simulink model "QuadcopterPID_Prop_Force_Thrust"  (R2026b)
settings: Solver=VariableStepAuto  StopTime=30  MaxStep=1e-2
undefined symbols (not defined in the file or in its folder): g, kT, M
libraries: slpidlib x1
settings Model: Creator=Aorus PC  LastModifiedBy=Ninad
settings OptimizationCC: ReuseModelBlockBuffer=off
settings SimscapeCC: SimscapeUseEnergyAccounting=off

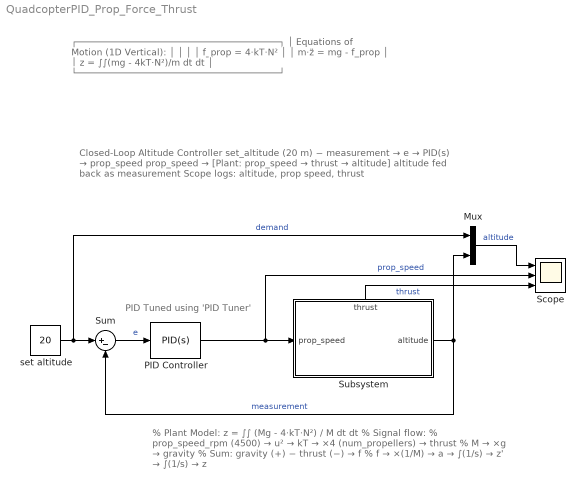
== system QuadcopterPID_Prop_Force_Thrust ==
  note: PID Tuned using 'PID Tuner'
  note: ┌──────────────────────────────────────┐
      | │  Equations of Motion (1D Vertical):  │
      | │                                      │
      | │  f_prop = 4·kT·N²                    │
      | │  m·z̈ = mg - f_prop                  │
      | │  z = ∫∫(mg - 4kT·N²)/m dt dt        │
      | └──────────────────────────────────────┘
  note: Closed-Loop Altitude Controller
      | set_altitude (20 m) − measurement → e → PID(s) → prop_speed
      | prop_speed → [Plant: prop_speed → thrust → altitude]
      | altitude fed back as measurement
      | Scope logs: altitude, prop speed, thrust
  note: % Plant Model: z = ∫∫ (Mg - 4·kT·N²) / M  dt dt
      | % Signal flow:
      | %   prop_speed_rpm (4500) → u² → kT → ×4 (num_propellers) → thrust
      | %   M → ×g → gravity
      | %   Sum: gravity (+) − thrust (−) → f
      | %   f → ×(1/M) → a → ∫(1/s) → z' → ∫(1/s) → z
  Mux : Mux  Inputs=2
  PID Controller : slpidlib/PID Controller  Controller=PID  Form=Parallel  TimeDomain=Continuous-time  UseExternalTs=off  SampleTime=-1  IntegratorMethod=Forward Euler  FilterMethod=Forward Euler  ControllerParametersSource=internal  P=200  I=50  UseKiTs=off  D=150  UseExternalDerivativeSource=off  N=10  UseFilter=on  TunerSelectOption=Transfer Function Based (PID Tuner App)  InitialConditionSource=internal  InitialConditionForIntegrator=4500  InitialConditionForFilter=0  DifferentiatorICPrevScaledInput=0  ExternalReset=none  TrackingMode=off  Kt=1  LimitOutput=on  SatLimitsSource=internal  UpperSaturationLimit=1e4  LowerSaturationLimit=0  LinearizeAsGain=on  AntiWindupMode=back-calculation  Kb=1  LimitIntegrator=on  UpperIntegratorSaturationLimit=1e4  LowerIntegratorSaturationLimit=0  POutMin=[]  POutMax=[]  IOutMin=[]  IOutMax=[]  DOutMin=[]  DOutMax=[]  NOutMin=[]  NOutMax=[]  SumOutMin=[]  SumOutMax=[]  SaturationOutMin=[]  SaturationOutMax=[]  PParamMin=[]  PParamMax=[]  IParamMin=[]  IParamMax=[]  DParamMin=[]  DParamMax=[]  NParamMin=[]  NParamMax=[]  KbParamMin=[]  KbParamMax=[]  KtParamMin=[]  KtParamMax=[]  KbOutMin=[]  KbOutMax=[]  KtOutMin=[]  KtOutMax=[]  IntegratorOutMin=[]  IntegratorOutMax=[]  FilterOutMin=[]  FilterOutMax=[]  SumI1OutMin=[]  SumI1OutMax=[]  SumI2OutMin=[]  SumI2OutMax=[]  SumI3OutMin=[]  SumI3OutMax=[]  SumI4OutMin=[]  SumI4OutMax=[]  SumDOutMin=[]  SumDOutMax=[]  DifferentiatorOutMin=[]  DifferentiatorOutMax=[]  FilterDiffOutCoefMin=[]  FilterDiffOutCoefMax=[]  ReciprocalOutMin=[]  ReciprocalOutMax=[]  SumDenOutMin=[]  SumDenOutMax=[]  SumNumOutMin=[]  SumNumOutMax=[]  DivideOutMin=[]  DivideOutMax=[]  UdiffTsProdOutMin=[]  UdiffTsProdOutMax=[]  NTsProdOutMin=[]  NTsProdOutMax=[]  UintegralTsProdOutMin=[]  UintegralTsProdOutMax=[]  UngainTsProdOutMin=[]  UngainTsProdOutMax=[]  ClampingZeroOutDataTypeStr=Inherit: Inherit via back propagation  ClampingZeroOutMin=[]  ClampingZeroOutMax=[]  FilterDenConstantOutDataTypeStr=Inherit: Inherit via back propagation  FilterDenConstantOutMin=[]  FilterDenConstantOutMax=[]  PCopyOutDataTypeStr=Inherit: Inherit via back propagation  PCopyOutMin=[]  PCopyOutMax=[]  NCopyOutDataTypeStr=Inherit: Inherit via back propagation  NCopyOutMin=[]  NCopyOutMax=[]  IntegratorContinuousStateAttributes=''  IntegratorStateMustResolveToSignalObject=off  IntegratorRTWStateStorageClass=Auto  FilterContinuousStateAttributes=''  FilterStateMustResolveToSignalObject=off  FilterRTWStateStorageClass=Auto  ParallelPVariant=InternalParameters  IdealPVariant=Disabled  IVariant=InternalParameters  DVariant=InternalParameters  IntegratorVariant=Continuous  SatVariant=Enabled  AWVariant=BackCalculation  PCopyVariant=Disabled  TRVariant=Disabled  FdbkBlocksVariant=Forward  IdealPFdbkVariant=Disabled  SatFdbkVariant=Disabled  DerivativeFilterVariant=ContFilter  NVariant=InternalParameters  NCopyVariant=Disabled  FilterICVariant=InternalICsFilter  IntegratorICVariant=InternalICs  ExternalResetVariant=Disabled  TRSumVariant=Passthrough  SumFdbkVariant=Disabled  SumVariant=Sum_PID  TsampFilterVariant=InternalTs  TsampNgainVariant=Passthrough  TsampIntegralVariant=Disabled_SignalSpec  ExternalSaturationOutDataTypeStr=Inherit: Same as second input  DerivativeSourceVariant=ErrorSignal  PreIntVariant=InternalPreInt
  Scope : Scope  NumInputPorts=3
      settings: ActiveDisplayYMinimum=-8.6140671509995883  ActiveDisplayYMaximum=29.721339228529466
  Subsystem : Subsystem
      settings: PortSchema="{\"entries\":[{\"content\":{\"sides\":[{\"content\":{\"connectorIds\":[\"In1\"]},\"type\":\"ConnectorPlacement.EquallySpacedRectSide\",\"uuid\":\"fbb4e32c-f4bd-454e-bff2-2681c96b2d03\"},{\"content\":{\"connectorIds\":[\"Out1\"],\"side\":\"RIGHT\"},\"type\":\"ConnectorPlacement.EquallySpacedRectSide\",\"uuid\":\"80437fec-448f-4d06-98df-4a328019d01a\"},{\"content\":{\"connectorIds\":[\"Out2\"],\"side\":\"TOP\"},\"type\":\"ConnectorPlacement.EquallySpacedRectSide\",\"uuid\":\"334ddea1-d867-47f1-b70d-72e605728c88\"}]},\"type\":\"ConnectorPlacement.EquallySpacedConnector\",\"uuid\":\"768cd58f-a8b0-4cb9-8b5d-1672039c996a\"}],\"packageUris\":[\"http://schema.mathworks.com/mf0/Connector/R2020b\"],\"version\":\"1.0\"}"
  Sum : Sum  Inputs=|+-
  set altitude : Constant  Value=20
  wires:
  PID Controller/1 -> Scope/2, Subsystem/1(prop_speed)  "prop_speed"
  Subsystem/1(altitude) -> Sum/2, Mux/2  "measurement"
  set altitude/1 -> Mux/1, Sum/1  "demand"
  Sum/1 -> PID Controller/1  "e"
  Mux/1 -> Scope/1  "altitude"
  Subsystem/2(thrust) -> Scope/3  "thrust"

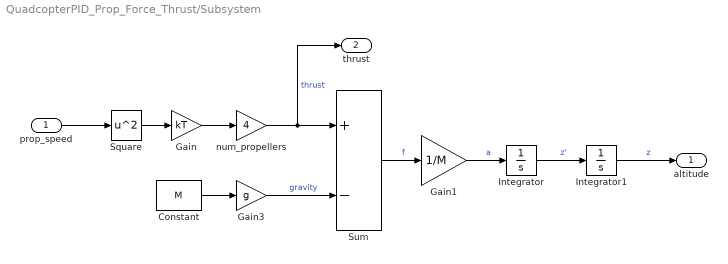
== system QuadcopterPID_Prop_Force_Thrust/Subsystem ==
  prop_speed : Inport
  Constant : Constant  Value=M
  Gain : Gain  Gain=kT
  Gain1 : Gain  Gain=1/M
  Gain3 : Gain  Gain=g
  Integrator : Integrator
  Integrator1 : Integrator  LimitOutput=on  LowerSaturationLimit=0
  Square : Math  Operator=square
  Sum : Sum  Inputs=+-
  num_propellers : Gain  Gain=4
  altitude : Outport
  thrust : Outport  Port=2
  wires:
  Integrator1/1 -> altitude/1  "z"
  Constant/1 -> Gain3/1
  num_propellers/1 -> thrust/1, Sum/1  "thrust"
  Square/1 -> Gain/1
  Gain1/1 -> Integrator/1  "a"
  Integrator/1 -> Integrator1/1  "z'"
  Sum/1 -> Gain1/1  "f"
  Gain3/1 -> Sum/2  "gravity"
  Gain/1 -> num_propellers/1
  prop_speed/1 -> Square/1
